simulink model "AEB_Project"  (R2024b)
settings: Solver=VariableStepAuto  StartTime=0.0  StopTime=5  RelTol=1e-3
libraries: simulink x3, slpidlib x1
settings Model: Creator=Hossam  LastModifiedBy=Hossam

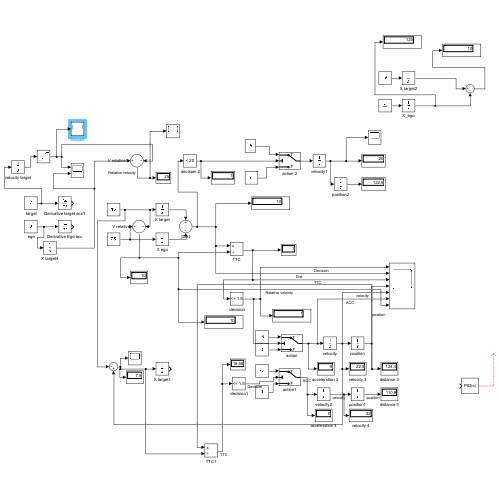
[thumbnail: Simulink's stored preview of the top-level diagram]
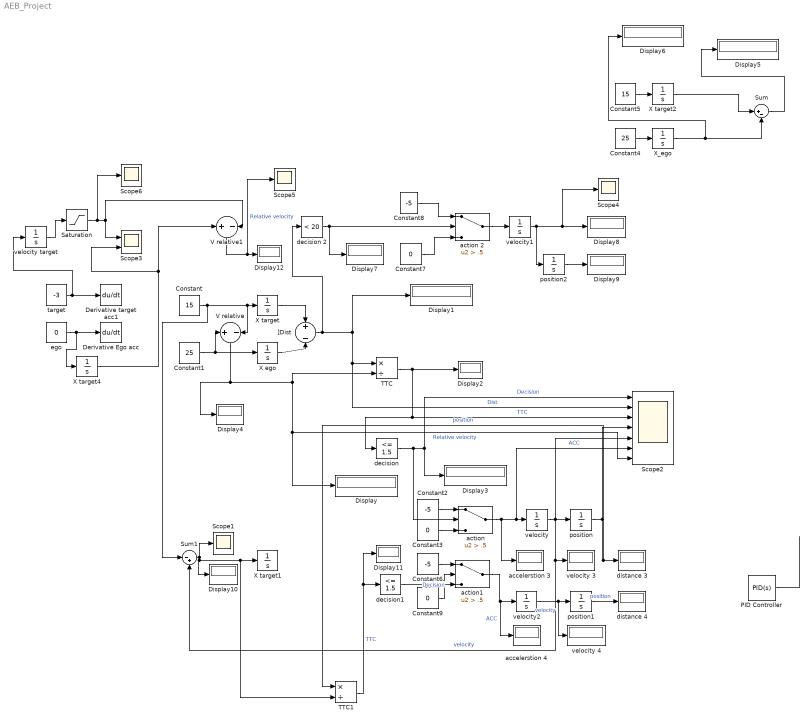
== system AEB_Project ==
  " decision" : simulink/Logic and Bit Operations/Compare To Constant  relop=<=  const=1.5  OutDataTypeStr=boolean
  " decision 2" : simulink/Logic and Bit Operations/Compare To Constant  relop=<  const=20  OutDataTypeStr=boolean
  " decision1" : simulink/Logic and Bit Operations/Compare To Constant  relop=<=  const=1.5  OutDataTypeStr=boolean
  " ego" : Constant  Value=0
  " target" : Constant  Value=-3
  Constant : Constant  Value=15
  Constant1 : Constant  Value=25
  Constant2 : Constant  Value=-5
  Constant3 : Constant  Value=0
  Constant4 : Constant  Value=25
  Constant5 : Constant  Value=15
  Constant6 : Constant  Value=-5
  Constant7 : Constant  Value=0
  Constant8 : Constant  Value=-5
  Constant9 : Constant  Value=0
  Derivative Ego acc : Derivative
  Derivative target acc1 : Derivative
  Display{,1..12} (13 alike) : Display
  PID Controller : slpidlib/PID Controller  Controller=PID  Form=Parallel  TimeDomain=Continuous-time  UseExternalTs=off  SampleTime=-1  IntegratorMethod=Forward Euler  FilterMethod=Forward Euler  ControllerParametersSource=internal  P=1  I=1  UseKiTs=off  D=0  UseExternalDerivativeSource=off  N=100  UseFilter=on  TunerSelectOption=Transfer Function Based (PID Tuner App)  InitialConditionSource=internal  InitialConditionForIntegrator=0  InitialConditionForFilter=0  DifferentiatorICPrevScaledInput=0  ExternalReset=none  TrackingMode=off  Kt=1  LimitOutput=off  SatLimitsSource=internal  UpperSaturationLimit=inf  LowerSaturationLimit=-inf  LinearizeAsGain=on  AntiWindupMode=none  Kb=1  LimitIntegrator=off  UpperIntegratorSaturationLimit=inf  LowerIntegratorSaturationLimit=-inf  POutMin=[]  POutMax=[]  IOutMin=[]  IOutMax=[]  DOutMin=[]  DOutMax=[]  NOutMin=[]  NOutMax=[]  SumOutMin=[]  SumOutMax=[]  SaturationOutMin=[]  SaturationOutMax=[]  PParamMin=[]  PParamMax=[]  IParamMin=[]  IParamMax=[]  DParamMin=[]  DParamMax=[]  NParamMin=[]  NParamMax=[]  KbParamMin=[]  KbParamMax=[]  KtParamMin=[]  KtParamMax=[]  KbOutMin=[]  KbOutMax=[]  KtOutMin=[]  KtOutMax=[]  IntegratorOutMin=[]  IntegratorOutMax=[]  FilterOutMin=[]  FilterOutMax=[]  SumI1OutMin=[]  SumI1OutMax=[]  SumI2OutMin=[]  SumI2OutMax=[]  SumI3OutMin=[]  SumI3OutMax=[]  SumI4OutMin=[]  SumI4OutMax=[]  SumDOutMin=[]  SumDOutMax=[]  DifferentiatorOutMin=[]  DifferentiatorOutMax=[]  FilterDiffOutCoefMin=[]  FilterDiffOutCoefMax=[]  ReciprocalOutMin=[]  ReciprocalOutMax=[]  SumDenOutMin=[]  SumDenOutMax=[]  SumNumOutMin=[]  SumNumOutMax=[]  DivideOutMin=[]  DivideOutMax=[]  UdiffTsProdOutMin=[]  UdiffTsProdOutMax=[]  NTsProdOutMin=[]  NTsProdOutMax=[]  UintegralTsProdOutMin=[]  UintegralTsProdOutMax=[]  UngainTsProdOutMin=[]  UngainTsProdOutMax=[]  ClampingZeroOutDataTypeStr=Inherit: Inherit via back propagation  ClampingZeroOutMin=[]  ClampingZeroOutMax=[]  FilterDenConstantOutDataTypeStr=Inherit: Inherit via back propagation  FilterDenConstantOutMin=[]  FilterDenConstantOutMax=[]  PCopyOutDataTypeStr=Inherit: Inherit via back propagation  PCopyOutMin=[]  PCopyOutMax=[]  NCopyOutDataTypeStr=Inherit: Inherit via back propagation  NCopyOutMin=[]  NCopyOutMax=[]  IntegratorContinuousStateAttributes=''  IntegratorStateMustResolveToSignalObject=off  IntegratorRTWStateStorageClass=Auto  FilterContinuousStateAttributes=''  FilterStateMustResolveToSignalObject=off  FilterRTWStateStorageClass=Auto  ParallelPVariant=InternalParameters  IdealPVariant=Disabled  IVariant=InternalParameters  DVariant=InternalParameters  IntegratorVariant=Continuous  SatVariant=Disabled  AWVariant=Passthrough  PCopyVariant=Disabled  TRVariant=Disabled  FdbkBlocksVariant=Forward  IdealPFdbkVariant=Disabled  SatFdbkVariant=Disabled  DerivativeFilterVariant=ContFilter  NVariant=InternalParameters  NCopyVariant=Disabled  FilterICVariant=InternalICsFilter  IntegratorICVariant=InternalICs  ExternalResetVariant=Disabled  TRSumVariant=Passthrough  SumFdbkVariant=Disabled  SumVariant=Sum_PID  TsampFilterVariant=InternalTs  TsampNgainVariant=Passthrough  TsampIntegralVariant=Disabled_SignalSpec  ExternalSaturationOutDataTypeStr=Inherit: Same as second input  DerivativeSourceVariant=ErrorSignal  PreIntVariant=InternalPreInt
  Saturation : Saturate  UpperLimit=15  LowerLimit=0
  Scope{1,4..6} (4 alike) : Scope
  Scope2 : Scope  NumInputPorts=7
  Scope3 : Scope  NumInputPorts=2
  Sum : Sum  Inputs=|+-
  Sum1 : Sum  Inputs=|-+
  TTC : Product  Inputs=*/
  TTC1 : Product  Inputs=*/
  V relative : Sum  Inputs=+-
  V relative1 : Sum  Inputs=+-
  X ego : Integrator
  X target : Integrator  InitialCondition=60
  X target1 : Integrator  InitialCondition=60
  X target2 : Integrator  InitialCondition=60
  X target4 : Integrator  InitialCondition=25
  X_ego : Integrator
  ]Dist : Sum  Inputs=+-
  "accelerstion 3 " : Display
  accelerstion 4 : Display
  action : Switch  Criteria=u2 > Threshold  Threshold=.5  SaturateOnIntegerOverflow=off  InputSameDT=off
  action 2 : Switch  Criteria=u2 > Threshold  Threshold=.5  SaturateOnIntegerOverflow=off  InputSameDT=off
  action1 : Switch  Criteria=u2 > Threshold  Threshold=.5  SaturateOnIntegerOverflow=off  InputSameDT=off
  distance 3 : Display
  distance 4 : Display
  position : Integrator
  position1 : Integrator
  position2 : Integrator
  velocity : Integrator  InitialCondition=25
  velocity 3 : Display
  velocity 4 : Display
  velocity target : Integrator  InitialCondition=15
  velocity1 : Integrator  InitialCondition=25
  velocity2 : Integrator  InitialCondition=25
  wires:
  Constant/1 -> X target/1, V relative/2, Sum1/1
  Constant1/1 -> X ego/1, V relative/1
  V relative/1 -> Display4/1, TTC/2, Display/1, Scope2/7  "Relative velocity"
  X target/1 -> ]Dist/1
  X ego/1 -> ]Dist/2
  ]Dist/1 -> " decision 2"/1, Scope2/2, TTC/1, Display1/1  "Dist"
  " decision"/1 -> action/2, Scope2/1, Display3/1  "Decision"
  Constant3/1 -> action/3
  Constant2/1 -> action/1
  action/1 -> "accelerstion 3 "/1, Scope2/6, velocity/1  "ACC"
  velocity/1 -> Sum1/2, velocity 3/1, Scope2/5, position/1  "velocity"
  position/1 -> Scope2/4, TTC1/1, distance 3/1  "position"
  Constant5/1 -> X target2/1
  Constant4/1 -> X_ego/1
  X target2/1 -> Sum/1
  X_ego/1 -> Display6/1, Sum/2
  Sum/1 -> Display5/1
  " decision 2"/1 -> action 2/2, Display7/1
  Constant8/1 -> action 2/1
  Constant7/1 -> action 2/3
  action 2/1 -> velocity1/1
  velocity1/1 -> Scope4/1, Display8/1, position2/1
  position2/1 -> Display9/1
  TTC/1 -> " decision"/1, Scope2/3, Display2/1  "TTC"
  Sum1/1 -> Scope1/1, TTC1/2, X target1/1, Display10/1
  TTC1/1 -> Display11/1, " decision1"/1  "TTC"
  " decision1"/1 -> action1/2  "Decision"
  Constant6/1 -> action1/1
  Constant9/1 -> action1/3
  action1/1 -> accelerstion 4/1, velocity2/1  "ACC"
  velocity2/1 -> velocity 4/1, position1/1  "velocity"
  position1/1 -> distance 4/1  "position"
  PID Controller/1 -> ?
  V relative1/1 -> Scope5/1, Display12/1  "Relative velocity"
  " target"/1 -> Derivative target acc1/1, velocity target/1
  " ego"/1 -> X target4/1, Derivative Ego acc/1
  velocity target/1 -> Saturation/1
  X target4/1 -> V relative1/1, Scope3/2
  Saturation/1 -> Scope6/1, V relative1/2, Scope3/1
